simulink model "youBot_Arm_before_acceleration_test"  (R2024a)
settings: Solver=ode15s  StartTime=0.0  StopTime=3.3  MaxStep=1e-2  RelTol=1e-3  AbsTol=1e-4
model workspace: external: MATLAB File youBot_DataFile.m (data not in the file)
undefined symbols (not defined in the file): Extr_Data_LinkHoles, Qt, sigbuilder_block, smiData, X, Y, YBT_Par, Z
libraries: sm_lib x193, nesl_utility x130, fl_lib x53, simulink x13, Parts_Lib x10, MyMath_lib x8, Motor_Lib x5, Contact_Forces_Lib x4, ee_lib x2, sdl_lib x2
(part 1 of 8)
CloseFcn:
  | try,close(h1_youBot_Arm),end
  | clear h1_youBot_Arm
  | try,close(h2_youBot_Arm),end
  | clear h2_youBot_Arm
  | try,close(h3_youBot_Arm),end
  | clear h3_youBot_Arm
  | try,close(h4_youBot_Arm),end
  | clear h4_youBot_Arm
  | try,close(h5_youBot_Arm),end
  | clear h5_youBot_Arm
  | 
  | try,close(h1_youbot_optim),end
  | clear h1_youbot_optim
  | try,close(h2_youbot_optim),end
  | clear h2_youbot_optim
  | try,close(h3_youbot_optim),end
  | clear h3_youbot_optim
  | try,close(h4_youbot_optim),end
  | clear h4_youbot_optim
  | 
  | 
  | clear simlog_youBot_Arm
  | clear logsout_simlog_youBot_Arm
Description:
  | youBot Arm
  | 
  | Copyright 2017-2024 The MathWorks, Inc.
settings Model: Creator=smiller  LastModifiedBy=ADMIN
settings SolverCC: AutoScaleAbsTol=off  AlgebraicLoopSolver=TrustRegion
settings DataIOCC: MaxDataPoints=15000  ReturnWorkspaceOutputs=off  SignalLoggingName=logsout_youBot_Arm
settings OptimizationCC: ReuseModelBlockBuffer=off
settings DebuggingCC: UnconnectedInputMsg=warning  UnconnectedOutputMsg=warning  UnconnectedLineMsg=warning  PregeneratedLibrarySubsystemCodeDiagnostic=none  ArithmeticOperatorsInVariantConditions=warning
settings ModelReferenceCC: EnableRefExpFcnMdlSchedulingChecks=on
settings SFSimCC: SimUseLocalCustomCode=off  CustomCodeUndefinedFunction=UseInterfaceOnly
settings RTWCC: RTWUseLocalCustomCode=off  GPUComputeCapability=3.5  DLArmComputeVersion=19.05
settings CodeAppCC: StateflowObjectComments=on
settings SimscapeCC: SimscapeNormalizeSystem=off  SimscapeLogType=all  SimscapeLogSimulationStatistics=on  SimscapeLogName=simlog_youBot_Arm  SimscapeLogLimitData=off  SimscapeLogDataHistory=15000
settings DiagnosticsConfigSet: SimMechanicsUnconnectedFramePorts=none  SimMechanicsUnconnectedGeometryPorts=none  SimMechanicsRigidlyBoundBlock=none
settings ExplorerConfigSet: InternalSimMechanicsExplorerSettings="<ExplorerConfiguration><canonicalview>default</canonicalview><AnimationSetting><BasePlaybackSpeed>1.0</BasePlaybackSpeed><PlaybackSpeedFactor>1.0</PlaybackSpeedFactor></AnimationSetting><TilePanel><TileInfo><Tiles Columns=\"1\" Count=\"1\" Rows=\"1\"><Column Left=\"2\" Weight=\"1\"/><Column Left=\"827\"/><Row Top=\"2\" Weight=\"1\"/><Row Top=\"551\"/><Tile Height=\"1\" Width=\"1\" X=\"0\" Y=\"0\"/></Tiles></TileInfo><SceneInfo><SceneViewer><BGColor><R>1</R><G>1</G><B>1</B></BGColor><Camera><DoPerspective>off</DoPerspective><Position><X>-0.83626486692763047</X><Y>0.83378966470538818</Y><Z>0.42271625808458047</Z></Position><Center><X>-0.12358625191225214</X><Y>0.13538177403089358</Y><Z>0.35702295596507261</Z></Center><Up><X>0.049916044320742092</X><Y>-0.042921475658829755</Y><Z>0.99783071482423225</Z></Up><ViewLimDist>1</ViewLimDist><YLim>0.36726038306951525</YLim><XLim>0.55497124552726751</XLim></Camera></SceneViewer></SceneInfo></TilePanel><MechEditorPanel><Cameras><Camera><Id>Camera1</Id><Value><Name>Box Rear</Name><NativeCamera><PositionTrackingFeature>Arm.Environment.Load.Box.Camera_Frames.Box_Rear.F</PositionTrackingFeature><CenterTrackingFeature>Arm.Environment.Load.Box.Camera_Frames.Box_Rear.F</CenterTrackingFeature><UpVectorTrackingFeature>Arm.Base.B</UpVectorTrackingFeature><CenterTrackingOrigin>off</CenterTrackingOrigin><CenterTrackingDirection>-Y</CenterTrackingDirection><UpVectorTrackingDirection>+Z</UpVectorTrackingDirection></NativeCamera></Value></Camera><Camera><Id>Camera2</Id><Value><Name>Box Right</Name><NativeCamera><PositionTrackingFeature>Arm.Environment.Load.Box.Camera_Frames.Box_Right.F</PositionTrackingFeature><CenterTrackingFeature>Arm.Environment.Load.Box.Camera_Frames.Box_Right.F</CenterTrackingFeature><UpVectorTrackingFeature>Arm.Base.B</UpVectorTrackingFeature><CenterTrackingOrigin>off</CenterTrackingOrigin><CenterTrackingDirection>+X</CenterTrackingDirection><UpVectorTrackingDirection>+Z</UpVectorTrackingDirection></NativeCamera></Value></Camera><Camera><Id>Camera3</Id><Value><Name>Box Left</Name><NativeCamera><PositionTrackingFeature>Arm.Environment.Load.Box.Camera_Frames.Box_Left.F</PositionTrackingFeature><CenterTrackingFeature>Arm.Environment.Load.Box.Camera_Frames.Box_Left.F</CenterTrackingFeature><UpVectorTrackingFeature>Arm.Base.B</UpVectorTrackingFeature><CenterTrackingOrigin>off</CenterTrackingOrigin><CenterTrackingDirection>-X</CenterTrackingDirection><UpVectorTrackingDirection>+Z</UpVectorTrackingDirection></NativeCamera></Value></Camera><Camera><Id>Camera4</Id><Value><Name>Flythrough</Name><NativeCamera><PositionKeyframeSet><Keyframe><Time>+0.0000000000000000e+00</Time><Value><X>-3.1054174760408881e-01</X><Y>+1.3491196588304544e+00</Y><Z>+3.2708238484160229e-01</Z></Value></Keyframe><Keyframe><Time>+2.2800000000000002e+00</Time><Value><X>-3.1054175822801983e-01</X><Y>+1.3491196588304541e+00</Y><Z>+3.2708238484160196e-01</Z></Value></Keyframe><Keyframe><Time>+5.1399999999999997e+00</Time><Value><X>-4.2421722692384516e-03</X><Y>+3.7992130540546115e-01</Y><Z>+2.9693194824033292e-01</Z></Value></Keyframe><Keyframe><Time>+6.3200000000000003e+00</Time><Value><X>-4.2421722692384516e-03</X><Y>+3.7992130540546115e-01</Y><Z>+2.9693194824033292e-01</Z></Value></Keyframe><Keyframe><Time>+6.9600000000000000e+00</Time><Value><X>+4.9536995356902480e-04</X><Y>+4.7137606352469363e-01</Y><Z>+9.0060852468013763e-02</Z></Value></Keyframe><Keyframe><Time>+9.0400000000000009e+00</Time><Value><X>-3.5306739807128906e-01</X><Y>+1.4091664089762709e-01</Y><Z>+7.5516276061534882e-02</Z></Value></Keyframe><Keyframe><Time>+1.1180000000000000e+01</Time><Value><X>-3.5306739807128906e-01</X><Y>+1.4091664089762709e-01</Y><Z>+7.5516276061534882e-02</Z></Value></Keyframe><Keyframe><Time>+1.3280000000000001e+01</Time><Value><X>-7.3703070570058815e-01</X><Y>+4.8587438383396610e-02</Y><Z>+1.0735257722565938e-01</Z></Value></Keyframe><Keyframe><Time>+1.4180000000000000e+01</Time><Value><X>-7.3703070570058815e-01</X><Y>+4.8587438383396610e-02</Y><Z>+1.0735257722565938e-01</Z></Value></Keyframe><Keyframe><Time>+1.6520000000000000e+01</Time><Value><X>-9.8573824482540429e-01</X><Y>+2.0670485208261197e-01</Y><Z>+2.1830120652472185e-01</Z></Value></Keyframe></PositionKeyframeSet><CenterKeyframeSet><Keyframe><Time>+0.0000000000000000e+00</Time><Value><X>-3.1054174760408881e-01</X><Y>+6.2094819104938748e-01</Y><Z>+3.2708238484160207e-01</Z></Value></Keyframe><Keyframe><Time>+2.2800000000000002e+00</Time><Value><X>-3.1054175822801983e-01</X><Y>+6.2094819104938725e-01</Y><Z>+3.2708238484160190e-01</Z></Value></Keyframe><Keyframe><Time>+5.1399999999999997e+00</Time><Value><X>-4.2448177918945106e-03</X><Y>+3.8051098782519893e-01</Y><Z>+5.9999998663807202e-02</Z></Value></Keyframe><Keyframe><Time>+6.3200000000000003e+00</Time><Value><X>-4.2448177918945106e-03</X><Y>+3.8051098782519893e-01</Y><Z>+5.9999998663807147e-02</Z></Value></Keyframe><Keyframe><Time>+6.9600000000000000e+00</Time><Value><X>+4.9536995356902480e-04</X><Y>+6.2306314706802368e-02</Y><Z>+9.0060852468013763e-02</Z></Value></Keyframe><Keyframe><Time>+9.0400000000000009e+00</Time><Value><X>-3.5306739807128906e-01</X><Y>+3.5937078297138214e-02</Y><Z>+7.5516276061534882e-02</Z></Value></Keyframe><Keyframe><Time>+1.1180000000000000e+01</Time><Value><X>-3.5306739807128906e-01</X><Y>+1.6846667071218728e-02</Y><Z>+7.5516276061534854e-02</Z></Value></Keyframe><Keyframe><Time>+1.3280000000000001e+01</Time><Value><X>-2.6908442378044128e-01</X><Y>+4.8587438383396610e-02</Y><Z>+1.0735257722565938e-01</Z></Value></Keyframe><Keyframe><Time>+1.4180000000000000e+01</Time><Value><X>-2.0696524530649185e-02</X><Y>+4.8587438383396610e-02</Y><Z>+1.0735257722565938e-01</Z></Value></Keyframe><Keyframe><Time>+1.6520000000000000e+01</Time><Value><X>-4.4591089802364647e-01</X><Y>+2.0670485208261191e-01</Y><Z>+2.1830120652472185e-01</Z></Value></Keyframe></CenterKeyframeSet><UpVectorKeyframeSet><Keyframe><Time>+0.0000000000000000e+00</Time><Value><X>+0.0000000000000000e+00</X><Y>-0.0000000000000000e+00</Y><Z>+1.0000000000000000e+00</Z></Value></Keyframe><Keyframe><Time>+2.2800000000000002e+00</Time><Value><X>+0.0000000000000000e+00</X><Y>-0.0000000000000000e+00</Y><Z>+1.0000000000000000e+00</Z></Value></Keyframe><Keyframe><Time>+5.1399999999999997e+00</Time><Value><X>-1.1959347625026685e-03</X><Y>-9.9999618779192856e-01</Y><Z>-2.4888032573367248e-03</Z></Value></Keyframe><Keyframe><Time>+6.3200000000000003e+00</Time><Value><X>-1.1959347625026687e-03</X><Y>-9.9999618779192878e-01</Y><Z>-2.4888032573366957e-03</Z></Value></Keyframe><Keyframe><Time>+6.9600000000000000e+00</Time><Value><X>+0.0000000000000000e+00</X><Y>-0.0000000000000000e+00</Y><Z>+1.0000000000000000e+00</Z></Value></Keyframe><Keyframe><Time>+9.0400000000000009e+00</Time><Value><X>+0.0000000000000000e+00</X><Y>-0.0000000000000000e+00</Y><Z>+1.0000000000000000e+00</Z></Value></Keyframe><Keyframe><Time>+1.1180000000000000e+01</Time><Value><X>+0.0000000000000000e+00</X><Y>-0.0000000000000000e+00</Y><Z>+1.0000000000000000e+00</Z></Value></Keyframe><Keyframe><Time>+1.3280000000000001e+01</Time><Value><X>+0.0000000000000000e+00</X><Y>+0.0000000000000000e+00</Y><Z>+1.0000000000000000e+00</Z></Value></Keyframe><Keyframe><Time>+1.4180000000000000e+01</Time><Value><X>+0.0000000000000000e+00</X><Y>+0.0000000000000000e+00</Y><Z>+1.0000000000000000e+00</Z></Value></Keyframe><Keyframe><Time>+1.6520000000000000e+01</Time><Value><X>+0.0000000000000000e+00</X><Y>+0.0000000000000000e+00</Y><Z>+1.0000000000000000e+00</Z></Value></Keyframe></UpVectorKeyframeSet></NativeCamera></Value></Camera></Cameras><GfxPanelCameraMap/><VideoCreator><PlaybackSpeedRatio>1.0</PlaybackSpeedRatio><FrameRate>30</FrameRate><VideoFormat>MPEG-4</VideoFormat><FrameSize>auto</FrameSize></VideoCreator></MechEditorPanel></ExplorerConfiguration>"

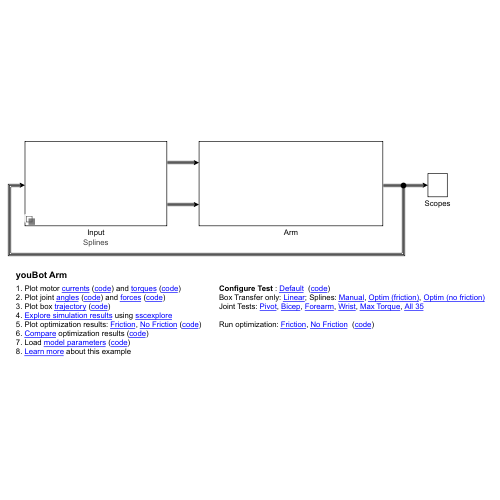
[thumbnail: Simulink's stored preview of the top-level diagram]
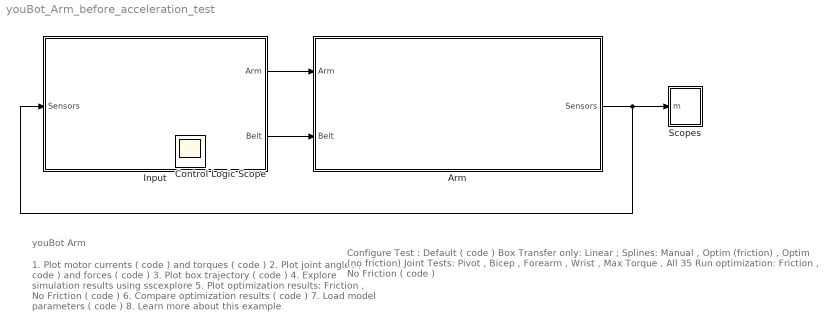
== system youBot_Arm_before_acceleration_test ==
  note: youBot Arm
  note: 1. Plot motor currents ( code ) and torques ( code )
      | 2. Plot joint angles ( code ) and forces ( code )
      | 3. Plot box trajectory ( code )
      | 4. Explore simulation results using sscexplore
      | 5. Plot optimization results: Friction , No Friction ( code )
      | 6. Compare optimization results ( code )
      | 7. Load model parameters ( code )
      | 8. Learn more about this example
  note: Configure Test : Default ( code )
      | Box Transfer only: Linear ; Splines: Manual , Optim (friction) , Optim (no friction)
      | Joint Tests: Pivot , Bicep , Forearm , Wrist , Max Torque , All 35
      |
      | Run optimization: Friction , No Friction ( code )
  Arm : Subsystem
      mask Display: image('youBot_Arm_System_IMAGE.jpg');
  Input : Subsystem  Tag=PublishSubsystem  Variant=on  VariantControlMode=label  VariantControl=Variant1  LabelModeActiveChoice=Splines
      settings: AttributesFormatString=%<ActiveVariant>
      mask Display:
      | blk = youBot_Arm_activeVariantBlock(gcb);
      | eval(get_param(blk, 'MaskDisplay'));
  Scopes : Subsystem
  Control Logic Scope : Scope
  wires:
  Input/1(Arm) -> Arm/1(Arm)
  Input/2(Belt) -> Arm/2(Belt)
  Arm/1(Sensors) -> Scopes/1(m), Input/1(Sensors)

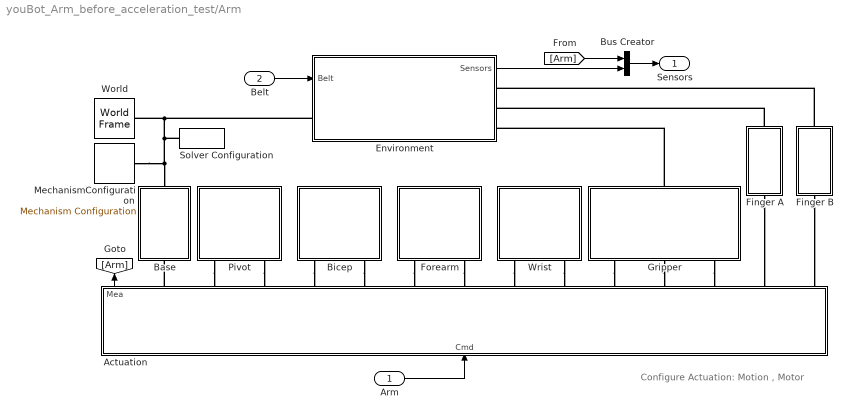
== system youBot_Arm_before_acceleration_test/Arm ==
  note: Configure Actuation: Motion , Motor
  Arm : Inport
  Belt : Inport  Port=2
  Actuation : Subsystem  Variant=on  VariantControlMode=label  LabelModeActiveChoice=Motion
      settings: AttributesFormatString=%<ActiveVariant>
      mask Display:
      | blk = youBot_Arm_activeVariantBlock(gcb);
      | eval(get_param(blk, 'MaskDisplay'));
  Base : Subsystem
      mask Display:
      | image('youBot_Arm_Base_IMAGE.jpg');
      | text(0.4,0.75,get_param(gcb,'Name'));
  Bicep : Subsystem
      mask Display:
      | image('youBot_Arm_Bicep_IMAGE.jpg');
      | text(0.6,0.9,get_param(gcb,'Name'));
  Bus Creator : BusCreator  Inputs=2
  Environment : Subsystem  Tag=PublishSubsystem
      mask Display: image('youBot_Arm_Environment_IMAGE.jpg');
  Finger A : Subsystem
      mask Display: image('youBot_Arm_Finger_A_IMAGE.jpg');
  Finger B : Subsystem
      mask Display: image('youBot_Arm_Finger_B_IMAGE.jpg');
  Forearm : Subsystem
      mask Display:
      | image('youBot_Arm_Forearm_IMAGE.jpg');
      | text(0.4,0.9,get_param(gcb,'Name'));
  Gripper : Subsystem
      mask Display:
      | image('youBot_Arm_Gripper_IMAGE.jpg');
      | text(0.6,0.9,'Gripper')
  MechanismConfiguration : sm_lib/Utilities/Mechanism Configuration  UniformGravity=Constant  GravityVector=[0 0 -9.81]  GravityVectorUnits=m/s^2  LinearizationDelta=0.001  JointModeTransitionNonlinearIterations=2
  Pivot : Subsystem
      mask Display:
      | image('youBot_Arm_Pivot_IMAGE.jpg');
      | text(0.6,0.9,get_param(gcb,'Name'));
  Solver Configuration : nesl_utility/Solver Configuration  PhysicalDomain=network_engine_domain  SubClassName=solver  LeftPortType=input  RightPortType=generic  Tones=[]  Harmonics=[]  SimulateNoise=off  Profile=off  UseLocalSampling=off  EnableSwitchedLinearOptims=on  FrequencyDomain=off  UseCCode=off  RelTol=0.001  AbsTol=1e-06  MinStep=1e-09  ToWorkspace=off  RevertToSquareIcSolve=off  NumHomotopyIterations=100  PhasorMode=off  PhasorModeNumHarmonics=1  ConsistencySolver=NEWTON_FTOL  IndexReductionMethod=DerivativeReplacement  DoDC=off  ResidualTolerance=1e-09  ConsistencyTolSource=GLOBAL  ConsistencyAbsTol=0.001  ConsistencyRelTol=0.001  ConsistencyTolFactor=0.001  UseLocalSolver=off  LocalSolverChoice=NE_BACKWARD_EULER_ADVANCER  ResolveIndetEquations=on  FunctionEvalNumThread=1  LocalSolverSampleTime=0.001  DoFixedCost=off  MaxNonlinIter=3  MaxModeIter=2  ComputeImpulses=off  ImpulseIterations=2  LinearAlgebra=Sparse  LinearAlgebraNumThread=0  EquationFormulation=NE_TIME_EF  DelaysMemoryBudget=1024  AutomaticFiltering=on  FilteringTimeConstant=0.001  PartitionStorageMethod=AS_NEEDED  PartitionMemoryBudget=1024  PartitionMethod=FAST  MultibodyUseLocalSolver=off  MultibodyLocalSolverChoice=ODE1  MultibodyLocalSolverSampleTime=0.001
  World : sm_lib/Frames and Transforms/World Frame
  Wrist : Subsystem
      mask Display:
      | image('youBot_Arm_Wrist_IMAGE.jpg');
      | text(0.6,0.9,get_param(gcb,'Name'));
  Sensors : Outport  VectorParamsAs1DForOutWhenUnconnected=off
  wires:
  Arm/1 -> Actuation/1(Cmd)
  Actuation/1(Mea) -> [Arm]
  Belt/1 -> Environment/1(Belt)
  Environment/1(Sensors) -> Bus Creator/2
  [Arm] -> Bus Creator/1
  Bus Creator/1 -> Sensors/1
  connections:
  Pivot/RConn1 -- Actuation/RConn2
  Wrist/RConn3 -- Actuation/RConn9
  Forearm/RConn1 -- Actuation/RConn6
  Forearm/RConn3 -- Actuation/RConn7
  Wrist/RConn1 -- Actuation/RConn8
  Pivot/RConn3 -- Actuation/RConn3
  Bicep/RConn1 -- Actuation/RConn4
  Bicep/RConn3 -- Actuation/RConn5
  Gripper/RConn1 -- Actuation/RConn10
  Finger A/LConn1 -- Actuation/RConn13
  Gripper/RConn3 -- Actuation/RConn12
  Gripper/RConn2 -- Actuation/RConn11
  Finger B/LConn1 -- Actuation/RConn14
  Actuation/RConn1 -- Base/RConn1
  MechanismConfiguration/RConn1 -- Environment/LConn1 -- World/RConn1 -- Solver Configuration/RConn1 -- Base/LConn1
  Finger B/RConn1 -- Environment/RConn1
  Finger A/RConn1 -- Environment/RConn2
  Gripper/LConn1 -- Environment/RConn3

== system youBot_Arm_before_acceleration_test/Input ==
  Sensors : Inport
  Control : Subsystem  VariantControl=Control
      mask Display:
      | image('youBot_Arm_Input_Control_IMAGE.jpg');
      | text(0.43,0.7,'Home');
      | text(0.235,0.32,'Belt In');
      | text(0.59,0.32,'Belt Out');
  Control Belt : Subsystem  VariantControl=Control_Belt
      mask Display:
      | image('youBot_Arm_Input_Control_Belt_IMAGE.jpg');
      | text(0.44,0.26,'Belts');
  Signals : Subsystem  VariantControl=Signals
      mask Display:
      | image('youBot_Arm_Input_Signals_IMAGE.jpg');
      | [~, activeGroupLabel]= signalbuilder([bdroot '/Input/Signals/Robot Commands'], 'activegroup');
      | text(0.25,0.5,activeGroupLabel);
  Splines : Subsystem  VariantControl=Splines
      mask Display: image('youBot_Arm_Input_Splines_IMAGE.jpg');
  Arm : Outport  VectorParamsAs1DForOutWhenUnconnected=off
  Belt : Outport  Port=2  VectorParamsAs1DForOutWhenUnconnected=off

== system youBot_Arm_before_acceleration_test/Scopes ==
  m : Inport
  Bus Selector : BusSelector  OutputSignals=Arm.P.t,Arm.B.t,Arm.F.t,Arm.W.t,Arm.G.t,Arm.a.f,Arm.b.f
  Bus Selector1 : BusSelector  OutputSignals=Arm.P.i,Arm.B.i,Arm.F.i,Arm.W.i,Arm.G.i,Arm.a.i,Arm.b.i
  Calculate Electrical Cost : Subsystem
  Calculate Torque Cost : Subsystem
  Currents : Scope  NumInputPorts=7
  Display : Display
  Display1 : Display
  Logging : Subsystem
  Mux : Mux
  Mux1 : Mux  Inputs=7
  Selector : Selector  InputPortWidth=7  IndexOptions=Index vector (dialog)  Indices=[1:4]  OutputSizes=1
  Terminator : Terminator
  Terminator1 : Terminator
  Torques : Scope  NumInputPorts=7
  wires:
  m/1 -> Bus Selector/1, Bus Selector1/1, Logging/1(In1)
  Bus Selector/1 -> Mux/1, Torques/1  "<t>"
  Bus Selector/2 -> Mux/2, Torques/2  "<t>"
  Bus Selector/4 -> Mux/4, Torques/4  "<t>"
  Bus Selector/7 -> Torques/7  "<f>"
  Bus Selector/3 -> Mux/3, Torques/3  "<t>"
  Bus Selector/5 -> Torques/5  "<t>"
  Bus Selector/6 -> Torques/6  "<f>"
  Mux/1 -> Calculate Torque Cost/1(x)
  Calculate Torque Cost/1(Int(x'*x)) -> Display/1, Terminator/1
  Bus Selector1/5 -> Mux1/5, Currents/5  "<i>"
  Bus Selector1/6 -> Mux1/6, Currents/6  "<i>"
  Bus Selector1/7 -> Mux1/7, Currents/7  "<i>"
  Bus Selector1/3 -> Mux1/3, Currents/3  "<i>"
  Bus Selector1/2 -> Mux1/2, Currents/2  "<i>"
  Bus Selector1/1 -> Mux1/1, Currents/1  "<i>"
  Bus Selector1/4 -> Mux1/4, Currents/4  "<i>"
  Mux1/1 -> Selector/1
  Calculate Electrical Cost/1(Int(x'*x)) -> Terminator1/1, Display1/1
  Selector/1 -> Calculate Electrical Cost/1(i)

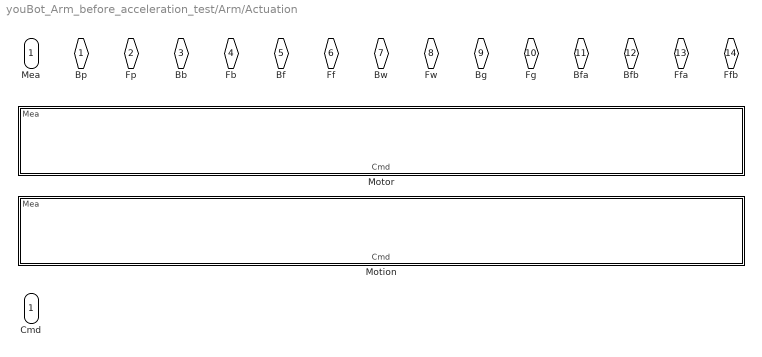
== system youBot_Arm_before_acceleration_test/Arm/Actuation ==
  Cmd : Inport
  Motion : Subsystem  Tag=PublishSubsystem  VariantControl=Motion
      mask Display: image('youBot_Arm_Actuation_Motion_IMAGE.jpg');
  Motor : Subsystem  Tag=PublishSubsystem  VariantControl=Motor
      mask Display: image('youBot_Arm_Actuation_Motor_IMAGE.jpg');
  Bp : PMIOPort  Side=Right
  Fp : PMIOPort  Port=2  Side=Right
  Bb : PMIOPort  Port=3  Side=Right
  Fb : PMIOPort  Port=4  Side=Right
  Bf : PMIOPort  Port=5  Side=Right
  Ff : PMIOPort  Port=6  Side=Right
  Bw : PMIOPort  Port=7  Side=Right
  Fw : PMIOPort  Port=8  Side=Right
  Bg : PMIOPort  Port=9  Side=Right
  Fg : PMIOPort  Port=10  Side=Right
  Bfa : PMIOPort  Port=11  Side=Right
  Bfb : PMIOPort  Port=12  Side=Right
  Ffa : PMIOPort  Port=13  Side=Right
  Ffb : PMIOPort  Port=14  Side=Right
  Mea : Outport  VectorParamsAs1DForOutWhenUnconnected=off

== system youBot_Arm_before_acceleration_test/Arm/Base ==
  Base_1_RIGID : Subsystem
  Transform : sm_lib/Frames and Transforms/Rigid Transform  RotationMethod=ArbitraryAxis  FollAlignAxisA=+X  BaseAlignAxisA=+Y  FollAlignAxisB=+Y  BaseAlignAxisB=+Z  RotationStandardAxis=+Z  RotationAngle=smiData.RigidTransform(49).angle  RotationAngleUnits=rad  RotationArbitraryAxis=smiData.RigidTransform(49).axis  RotationSequenceAxes=FollowerAxes  RotationSequence=XYX  RotationSequenceAngles=[0 0 0]  RotationSequenceAnglesUnits=deg  RotationMatrix=[1 0 0; 0 1 0; 0 0 1]  Quaternion=[1 0 0 0]  TranslationMethod=Cartesian  TranslationCartesianOffset=smiData.RigidTransform(49).translation  TranslationCartesianOffsetUnits=m  TranslationStandardAxis=+Z  TranslationStandardOffset=0  TranslationStandardOffsetUnits=m  TranslationROffset=0  TranslationROffsetUnits=m  TranslationThetaOffset=0  TranslationThetaOffsetUnits=deg  TranslationZOffset=0  TranslationZOffsetUnits=m
  B : PMIOPort  Side=Left
  F : PMIOPort  Port=2  Side=Right
  connections:
  Base_1_RIGID/RConn1 -- F/RConn1
  Transform/LConn1 -- B/RConn1
  Base_1_RIGID/LConn1 -- Transform/RConn1

== system youBot_Arm_before_acceleration_test/Arm/Bicep ==
  note: Connection 2 added only to adjust position of subsystem ports.
  Bicep_1_RIGID : Subsystem
  B : PMIOPort  Side=Right
  ~ : PMIOPort  Tag=CustomStyle  Port=2  Side=Right
  F : PMIOPort  Port=3  Side=Right
  connections:
  Bicep_1_RIGID/LConn1 -- B/RConn1
  ~/RConn1 -- Bicep_1_RIGID/RConn1 -- F/RConn1

== system youBot_Arm_before_acceleration_test/Arm/Environment ==
  note: Configure Load: Payload , Damper , Penalty
  Belt : Inport
  Conveyors : Subsystem
      mask Display: image('youBot_Arm_Conveyors_IMAGE.jpg');
  EE Signals : Subsystem
  Floor : Subsystem
  Gripper Force : Subsystem  Tag=PublishSubsystem  Variant=on  VariantControlMode=label  LabelModeActiveChoice=Payload
      settings: AttributesFormatString=%<ActiveVariant>
      mask Display:
      | blk = youBot_Arm_activeVariantBlock(gcb);
      | eval(get_param(blk, 'MaskDisplay'));
  Load : Subsystem  Variant=on  VariantControlMode=label  LabelModeActiveChoice=None
      settings: AttributesFormatString=%<ActiveVariant>
      mask Display:
      | blk = youBot_Arm_activeVariantBlock(gcb);
      | eval(get_param(blk, 'MaskDisplay'));
  To Workspace : ToWorkspace  VariableName=EE_xyz  SaveFormat=Structure With Time  SampleTime=-1
  Transform Sensor EE : sm_lib/Frames and Transforms/Transform Sensor  MeasurementFrame=World  RotationSequence=XYX  SenseAngle=off  SenseAxis=off  SenseQ=off  SenseR=off  SenseRotationSequence=off  SenseOmegaX=off  SenseOmegaY=off  SenseOmegaZ=off  SenseOmega=off  SenseQDot=off  SenseRDot=off  SenseRotationSequenceDot=off  SenseAlphaX=off  SenseAlphaY=off  SenseAlphaZ=off  SenseAlpha=off  SenseQDDot=off  SenseRDDot=off  SenseX=on  SenseY=on  SenseZ=on  SenseXYZ=off  SenseRad=off  SenseAzim=off  SenseDist=off  SenseInc=off  SenseXDot=off  SenseYDot=off  SenseZDot=off  SenseXYZDot=off  SenseRadDot=off  SenseAzimDot=off  SenseDistDot=off  SenseIncDot=off  SenseXDDot=off  SenseYDDot=off  SenseZDDot=off  SenseXYZDDot=off  SenseRadDDot=off  SenseAzimDDot=off  SenseDistDDot=off  SenseIncDDot=off
  W : PMIOPort  Side=Left
  Fb : PMIOPort  Port=2  Side=Right
  Fa : PMIOPort  Port=3  Side=Right
  E : PMIOPort  Port=4  Side=Right
  Sensors : Outport  VectorParamsAs1DForOutWhenUnconnected=off
  wires:
  EE Signals/1(xyz) -> To Workspace/1
  Belt/1 -> Conveyors/1(Belt)
  Conveyors/1(Sensors) -> Sensors/1
  connections:
  Gripper Force/RConn1 -- Fa/RConn1
  Gripper Force/LConn1 -- Load/RConn1
  Gripper Force/RConn3 -- Fb/RConn1
  Gripper Force/LConn2 -- Load/RConn2
  Gripper Force/RConn2 -- Transform Sensor EE/RConn1 -- E/RConn1
  EE Signals/LConn1 -- Transform Sensor EE/RConn2
  EE Signals/LConn2 -- Transform Sensor EE/RConn3
  EE Signals/LConn3 -- Transform Sensor EE/RConn4
  Load/LConn1 -- Conveyors/RConn1
  Load/LConn2 -- Transform Sensor EE/LConn1 -- Floor/LConn1 -- W/RConn1 -- Conveyors/LConn1

== system youBot_Arm_before_acceleration_test/Arm/Finger A ==
  Finger_A_1_RIGID : Subsystem
  F : PMIOPort  Side=Left
  f : PMIOPort  Port=2  Side=Right
  connections:
  f/RConn1 -- Finger_A_1_RIGID/RConn1
  F/RConn1 -- Finger_A_1_RIGID/LConn1

== system youBot_Arm_before_acceleration_test/Arm/Finger B ==
  Finger_B_1_RIGID : Subsystem
  F : PMIOPort  Side=Left
  f : PMIOPort  Port=2  Side=Right
  connections:
  f/RConn1 -- Finger_B_1_RIGID/RConn1
  Finger_B_1_RIGID/LConn1 -- F/RConn1

== system youBot_Arm_before_acceleration_test/Arm/Forearm ==
  note: Connection 2 added only to adjust position of subsystem ports.
  Forearm_1_RIGID : Subsystem
  Forearm_Black_Inlay_1_RIGID : Subsystem
  B : PMIOPort  Side=Right
  ~ : PMIOPort  Port=2  Side=Right
  F : PMIOPort  Port=3  Side=Right
  connections:
  Forearm_1_RIGID/LConn2 -- B/RConn1
  ~/RConn1 -- Forearm_1_RIGID/RConn1 -- F/RConn1
  Forearm_1_RIGID/LConn1 -- Forearm_Black_Inlay_1_RIGID/LConn1

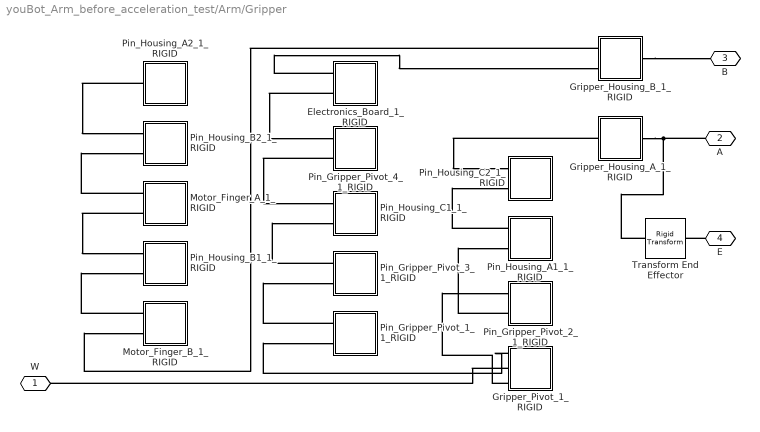
== system youBot_Arm_before_acceleration_test/Arm/Gripper ==
  Electronics_Board_1_RIGID : Subsystem
  Gripper_Housing_A_1_RIGID : Subsystem
  Gripper_Housing_B_1_RIGID : Subsystem
  Gripper_Pivot_1_RIGID : Subsystem
  Motor_Finger_A_1_RIGID : Subsystem
  Motor_Finger_B_1_RIGID : Subsystem
  Pin_Gripper_Pivot_1_1_RIGID : Subsystem
  Pin_Gripper_Pivot_2_1_RIGID : Subsystem
  Pin_Gripper_Pivot_3_1_RIGID : Subsystem
  Pin_Gripper_Pivot_4_1_RIGID : Subsystem
  Pin_Housing_A1_1_RIGID : Subsystem
  Pin_Housing_A2_1_RIGID : Subsystem
  Pin_Housing_B1_1_RIGID : Subsystem
  Pin_Housing_B2_1_RIGID : Subsystem
  Pin_Housing_C1_1_RIGID : Subsystem
  Pin_Housing_C2_1_RIGID : Subsystem
  Transform End Effector : sm_lib/Frames and Transforms/Rigid Transform  RotationMethod=AlignedAxes  FollAlignAxisA=+Z  BaseAlignAxisA=-Z  FollAlignAxisB=+X  BaseAlignAxisB=+Y  RotationStandardAxis=+Z  RotationAngle=0.0  RotationAngleUnits=deg  RotationArbitraryAxis=[0 0 1]  RotationSequenceAxes=FollowerAxes  RotationSequence=XYX  RotationSequenceAngles=[0 0 0]  RotationSequenceAnglesUnits=deg  RotationMatrix=[1 0 0; 0 1 0; 0 0 1]  Quaternion=[1 0 0 0]  TranslationMethod=StandardAxis  TranslationCartesianOffset=[0 0 0]  TranslationCartesianOffsetUnits=m  TranslationStandardAxis=+X  TranslationStandardOffset=YBT_Par.Payload.gripper_ref_offset  TranslationStandardOffsetUnits=m  TranslationROffset=0  TranslationROffsetUnits=m  TranslationThetaOffset=0  TranslationThetaOffsetUnits=deg  TranslationZOffset=0  TranslationZOffsetUnits=m
  W : PMIOPort  Side=Right
  A : PMIOPort  Port=2  Side=Right
  B : PMIOPort  Port=3  Side=Right
  E : PMIOPort  Port=4  Side=Left
  connections:
  Gripper_Housing_B_1_RIGID/RConn1 -- B/RConn1
  A/RConn1 -- Gripper_Housing_A_1_RIGID/RConn1 -- Transform End Effector/LConn1
  E/RConn1 -- Transform End Effector/RConn1
  Pin_Gripper_Pivot_1_1_RIGID/LConn1 -- Pin_Gripper_Pivot_3_1_RIGID/LConn2
  Pin_Housing_A2_1_RIGID/LConn1 -- Pin_Housing_B2_1_RIGID/LConn1
  Gripper_Pivot_1_RIGID/LConn2 -- W/RConn1
  Gripper_Pivot_1_RIGID/LConn3 -- Pin_Gripper_Pivot_2_1_RIGID/LConn1
  Gripper_Pivot_1_RIGID/LConn1 -- Pin_Gripper_Pivot_1_1_RIGID/LConn2
  Pin_Housing_A1_1_RIGID/LConn1 -- Pin_Housing_C2_1_RIGID/LConn2
  Gripper_Housing_A_1_RIGID/LConn1 -- Pin_Housing_C2_1_RIGID/LConn1
  Motor_Finger_A_1_RIGID/LConn2 -- Pin_Housing_B1_1_RIGID/LConn1
  Gripper_Housing_B_1_RIGID/LConn1 -- Motor_Finger_B_1_RIGID/LConn2
  Electronics_Board_1_RIGID/LConn2 -- Pin_Gripper_Pivot_4_1_RIGID/LConn1
  Motor_Finger_A_1_RIGID/LConn1 -- Pin_Housing_B2_1_RIGID/LConn2
  Pin_Gripper_Pivot_3_1_RIGID/LConn1 -- Pin_Housing_C1_1_RIGID/LConn2
  Electronics_Board_1_RIGID/LConn1 -- Gripper_Housing_B_1_RIGID/LConn2
  Pin_Gripper_Pivot_2_1_RIGID/LConn2 -- Pin_Housing_A1_1_RIGID/LConn2
  Pin_Gripper_Pivot_4_1_RIGID/LConn2 -- Pin_Housing_C1_1_RIGID/LConn1
  Motor_Finger_B_1_RIGID/LConn1 -- Pin_Housing_B1_1_RIGID/LConn2

== system youBot_Arm_before_acceleration_test/Arm/Pivot ==
  note: Connection 2 added only to adjust position of subsystem ports.
  Pivot_1_RIGID : Subsystem
  Pivot_Black_Inlay_1_RIGID : Subsystem
  B : PMIOPort  Side=Right
  ~ : PMIOPort  Tag=CustomStyle  Port=2  Side=Right
  F : PMIOPort  Port=3  Side=Right
  connections:
  Pivot_1_RIGID/LConn2 -- B/RConn1
  ~/RConn1 -- Pivot_1_RIGID/RConn1 -- F/RConn1
  Pivot_1_RIGID/LConn1 -- Pivot_Black_Inlay_1_RIGID/LConn1

== system youBot_Arm_before_acceleration_test/Arm/Wrist ==
  note: Connection 2 added only to adjust position of subsystem ports.
  Wrist_1_RIGID : Subsystem
  B : PMIOPort  Side=Right
  ~ : PMIOPort  Port=2  Side=Right
  F : PMIOPort  Port=3  Side=Right
  connections:
  F/RConn1 -- ~/RConn1 -- Wrist_1_RIGID/RConn1
  Wrist_1_RIGID/LConn1 -- B/RConn1

== system youBot_Arm_before_acceleration_test/Input/Control ==
  Sensors : Inport
  Bus Creator : BusCreator  Inputs=2
  Bus Selector : BusSelector  OutputSignals=Belts.BeltIn.Box,Belts.BeltIn.LC,Belts.BeltOut.Box,Belts.BeltOut.LC
  Joint Commands : Subsystem  mask{home2in=YBT_Par.Waypoints.Home2In.Manual, in2out=YBT_Par.Waypoints.In2Out.Manual, out2home=YBT_Par.Waypoints.Out2Home.Manual}
      mask prompts: home2in "Home to Belt In"; in2out "Belt In to Belt Out"; out2home "Belt Out to Home"
  Logging : Subsystem
  Logic : Stateflow chart  Tag=PublishSubsystem  TreatAsAtomicUnit=on  mask(Supervisory Logic for Arm, Gripper, and Belts){delayMoveBox=YBT_Par.Control.Logic.Delay_Move_Box, delayGripBox=YBT_Par.Control.Logic.Delay_Grip_Box, delayDropBox=YBT_Par.Control.Logic.Delay_Drop_Box, delayClose=YBT_Par.Control.Logic.Delay_Close_Grip, delayBeltClear=YBT_Par.Control.Logic.Delay_Belt_Clear, delayShipBox=YBT_Par.Control.Logic.Delay_Ship_Box}
      mask prompts: delayMoveBox "Delay Move Box (sec)"; delayGripBox "Delay Grip Box (sec)"; delayDropBox "Delay Drop Box (sec)"; delayClose "Delay Close Gripper at Home (sec)"; delayBeltClear "Delay Belt Clear (sec)"; delayShipBox "Delay Ship Box (sec)"
      mask help: Logic controlling robot arm, gripper, and belts. Arm movement, gripper state, and belt state are controlled based on events in the system. The parameters below are for delays that ensure actions are not triggered too early.
  Arm : Outport  VectorParamsAs1DForOutWhenUnconnected=off
  Belt : Outport  Port=2  VectorParamsAs1DForOutWhenUnconnected=off
  wires:
  Bus Creator/1 -> Belt/1
  Bus Selector/4 -> Logic/4(BeltOut_LC)  "<LC>"
  Bus Selector/3 -> Logic/3(BeltOut_Box)  "<Box>"
  Bus Selector/2 -> Logic/2(BeltIn_LC)  "<LC>"
  Bus Selector/1 -> Logic/1(BeltIn_Box)  "<Box>"
  Sensors/1 -> Logging/1(S), Bus Selector/1
  Logic/3(BeltIn_En) -> Bus Creator/1  "Belt In On"
  Logic/1(Way) -> Joint Commands/1(Way)  "Way"
  Logic/2(Grip) -> Joint Commands/2(Grip)  "Grip"
  Logic/4(BeltOut_En) -> Bus Creator/2  "Belt Out On"
  Joint Commands/1(bus) -> Arm/1

== system youBot_Arm_before_acceleration_test/Input/Control Belt ==
  Sensors : Inport
  Bus Creator : BusCreator  Inputs=2
  Bus Selector : BusSelector  OutputSignals=Belts.BeltIn.Box,Belts.BeltIn.LC,Belts.BeltOut.Box,Belts.BeltOut.LC
  Control Belt In : Subsystem
  Control Belt Out : Subsystem
  Robot Commands : Subsystem  Tag=STV Subsys  LoadFcn=sigbuilder_block('load');  StartFcn=sigbuilder_block('start');  StopFcn=sigbuilder_block('stop');  ClipboardFcn=sigbuilder_block('clipboard');  mask(Sigbuilder block){tuvar=[0:10]}
      mask help: Simulink:masks:SigbuilderBlock_MD
      mask init:
      | if ~strcmp(get_param(bdroot(gcbh),'SimulationStatus'),'stopped') tuvar = sigbuilder_block('maskInit'); end
      settings: CopyFcn=sigbuilder_block('copy');  DeleteFcn=sigbuilder_block('delete');  ModelCloseFcn=sigbuilder_block('modelClose');  PreSaveFcn=sigbuilder_block('preSave');  PauseFcn=sigbuilder_block('pause');  ContinueFcn=sigbuilder_block('continue');  NameChangeFcn=sigbuilder_block('namechange');  OpenFcn=sigbuilder_block('open',[0 142.8 450.6 439.8 ]);  CloseFcn=sigbuilder_block('close');
      mask Display: plot(0, 0, 100, 100,[2, 2, 32, 32, 2], [68, 8, 8, 68, 68],[32, 2], [38, 38], [32, 19, 2],[53, 60, 44], [32, 17, 17, 2],[16, 16, 31, 31]);txt = getActiveGroup(gcbh);text(2, 100, txt,'verticalAlignment', 'top');
  Arm : Outport  VectorParamsAs1DForOutWhenUnconnected=off
  Belt : Outport  Port=2  VectorParamsAs1DForOutWhenUnconnected=off
  wires:
  Robot Commands/1(Bus) -> Arm/1
  Sensors/1 -> Bus Selector/1
  Bus Selector/1 -> Control Belt In/1(BeltOut)  "<Box>"
  Bus Selector/2 -> Control Belt In/2(Sensor)  "<LC>"
  Bus Selector/3 -> Control Belt Out/1(BeltOut)  "<Box>"
  Bus Selector/4 -> Control Belt Out/2(Sensor)  "<LC>"
  Control Belt In/1(On) -> Bus Creator/1  "Belt In On"
  Control Belt Out/1(On) -> Bus Creator/2  "Belt Out On"
  Bus Creator/1 -> Belt/1

== system youBot_Arm_before_acceleration_test/Input/Signals ==
  Belt Commands : Subsystem  Tag=STV Subsys  LoadFcn=sigbuilder_block('load');  StartFcn=sigbuilder_block('start');  StopFcn=sigbuilder_block('stop');  ClipboardFcn=sigbuilder_block('clipboard');  mask(Sigbuilder block){tuvar=[0:10]}
      mask help: Simulink:masks:SigbuilderBlock_MD
      mask init:
      | if ~strcmp(get_param(bdroot(gcbh),'SimulationStatus'),'stopped') tuvar = sigbuilder_block('maskInit'); end
      settings: CopyFcn=sigbuilder_block('copy');  DeleteFcn=sigbuilder_block('delete');  ModelCloseFcn=sigbuilder_block('modelClose');  PreSaveFcn=sigbuilder_block('preSave');  PauseFcn=sigbuilder_block('pause');  ContinueFcn=sigbuilder_block('continue');  NameChangeFcn=sigbuilder_block('namechange');  OpenFcn=sigbuilder_block('open',[19.2 172.2 550.8 400.2 ]);  CloseFcn=sigbuilder_block('close');
      mask Display: plot(0, 0, 100, 100,[2, 2, 32, 32, 2], [68, 8, 8, 68, 68],[32, 2], [38, 38], [32, 19, 2],[53, 60, 44], [32, 17, 17, 2],[16, 16, 31, 31]);txt = getActiveGroup(gcbh);text(2, 100, txt,'verticalAlignment', 'top');
  Robot Commands : Subsystem  Tag=STV Subsys  LoadFcn=sigbuilder_block('load');  StartFcn=sigbuilder_block('start');  StopFcn=sigbuilder_block('stop');  ClipboardFcn=sigbuilder_block('clipboard');  mask(Sigbuilder block){tuvar=[0:10]}
      mask help: Simulink:masks:SigbuilderBlock_MD
      mask init:
      | if ~strcmp(get_param(bdroot(gcbh),'SimulationStatus'),'stopped') tuvar = sigbuilder_block('maskInit'); end
      settings: CopyFcn=sigbuilder_block('copy');  DeleteFcn=sigbuilder_block('delete');  ModelCloseFcn=sigbuilder_block('modelClose');  PreSaveFcn=sigbuilder_block('preSave');  PauseFcn=sigbuilder_block('pause');  ContinueFcn=sigbuilder_block('continue');  NameChangeFcn=sigbuilder_block('namechange');  OpenFcn=sigbuilder_block('open',[0.6 142.2 450.6 439.8 ]);  CloseFcn=sigbuilder_block('close');
      mask Display: plot(0, 0, 100, 100,[2, 2, 32, 32, 2], [68, 8, 8, 68, 68],[32, 2], [38, 38], [32, 19, 2],[53, 60, 44], [32, 17, 17, 2],[16, 16, 31, 31]);txt = getActiveGroup(gcbh);text(2, 100, txt,'verticalAlignment', 'top');
  Arm : Outport  VectorParamsAs1DForOutWhenUnconnected=off
  Belt : Outport  Port=2  VectorParamsAs1DForOutWhenUnconnected=off
  wires:
  Robot Commands/1(Bus) -> Arm/1
  Belt Commands/1(Bus) -> Belt/1

== system youBot_Arm_before_acceleration_test/Input/Splines ==
  Bus Creator : BusCreator  Inputs=7
  Bus Creator3 : BusCreator  Inputs=2
  Clock : Clock
  Constant : Constant  Value=0
  Constant1 : Constant  Value=YBT_Par.Gripper.Position.tight
  Constant2 : Constant  Value=YBT_Par.Gripper.Position.tight
  Spline Bicep Angle : Lookup_n-D  NumberOfTableDimensions=1  LookupTableObject=''  BreakpointsForDimension1=t  Table=Qt(2,:)  InterpMethod=Cubic spline  ExtrapMethod=Clip  InternalRulePriority=Speed  RndMeth=Simplest
  Spline Forearm Angle : Lookup_n-D  NumberOfTableDimensions=1  LookupTableObject=''  BreakpointsForDimension1=t  Table=Qt(3,:)  InterpMethod=Cubic spline  ExtrapMethod=Clip  InternalRulePriority=Speed  RndMeth=Simplest
  Spline Pivot Angle : Lookup_n-D  NumberOfTableDimensions=1  LookupTableObject=''  BreakpointsForDimension1=t  Table=Qt(1,:)  InterpMethod=Cubic spline  ExtrapMethod=Clip  InternalRulePriority=Speed  RndMeth=Simplest
  Spline Wrist Angle : Lookup_n-D  NumberOfTableDimensions=1  LookupTableObject=''  BreakpointsForDimension1=t  Table=Qt(4,:)  InterpMethod=Cubic spline  ExtrapMethod=Clip  InternalRulePriority=Speed  RndMeth=Simplest
  vx : Constant  Value=0
  vy : Constant  Value=0
  Arm : Outport  VectorParamsAs1DForOutWhenUnconnected=off
  Belt : Outport  Port=2  VectorParamsAs1DForOutWhenUnconnected=off
  wires:
  Bus Creator/1 -> Arm/1
  Spline Pivot Angle/1 -> Bus Creator/1  "cP"
  Spline Bicep Angle/1 -> Bus Creator/2  "cB"
  Spline Forearm Angle/1 -> Bus Creator/3  "cF"
  Spline Wrist Angle/1 -> Bus Creator/4  "cW"
  Constant/1 -> Bus Creator/5  "cG"
  Constant1/1 -> Bus Creator/6  "ca"
  Constant2/1 -> Bus Creator/7  "cb"
  Clock/1 -> Spline Wrist Angle/1, Spline Forearm Angle/1, Spline Pivot Angle/1, Spline Bicep Angle/1
  vx/1 -> Bus Creator3/1  "Belt In On"
  vy/1 -> Bus Creator3/2  "Belt Out On"
  Bus Creator3/1 -> Belt/1

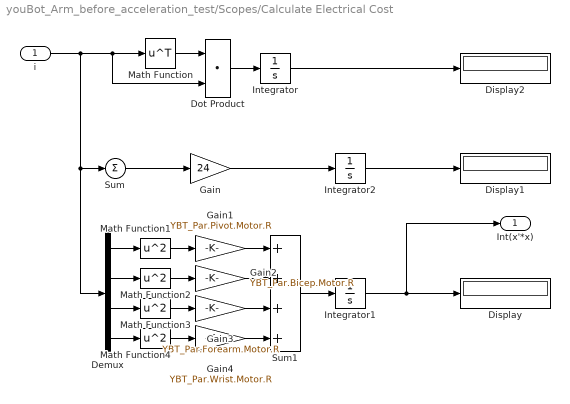
== system youBot_Arm_before_acceleration_test/Scopes/Calculate Electrical Cost ==
  i : Inport
  Demux : Demux
  Display : Display
  Display1 : Display
  Display2 : Display
  Dot Product : DotProduct  OutDataTypeStr=Inherit: Inherit via internal rule
  Gain : Gain  Gain=24
  Gain1 : Gain  Gain=YBT_Par.Pivot.Motor.R
  Gain2 : Gain  Gain=YBT_Par.Bicep.Motor.R
  Gain3 : Gain  Gain=YBT_Par.Forearm.Motor.R
  Gain4 : Gain  Gain=YBT_Par.Wrist.Motor.R
  Integrator : Integrator
  Integrator1 : Integrator
  Integrator2 : Integrator
  Math Function : Math  Operator=transpose  SignedPower=on
  Math Function{1..4} (4 alike) : Math  Operator=square  SignedPower=on
  Sum : Sum  Inputs=+
  Sum1 : Sum  Inputs=++++
  Int(x'*x) : Outport  VectorParamsAs1DForOutWhenUnconnected=off
  wires:
  Integrator/1 -> Display2/1
  i/1 -> Demux/1, Sum/1, Math Function/1, Dot Product/2
  Math Function/1 -> Dot Product/1
  Dot Product/1 -> Integrator/1
  Sum/1 -> Gain/1
  Demux/1 -> Math Function1/1
  Math Function1/1 -> Gain1/1
  Demux/2 -> Math Function2/1
  Math Function2/1 -> Gain2/1
  Demux/3 -> Math Function3/1
  Math Function3/1 -> Gain3/1
  Demux/4 -> Math Function4/1
  Math Function4/1 -> Gain4/1
  Gain1/1 -> Sum1/1
  Gain2/1 -> Sum1/2
  Gain3/1 -> Sum1/3
  Gain4/1 -> Sum1/4
  Sum1/1 -> Integrator1/1
  Gain/1 -> Integrator2/1
  Integrator1/1 -> Int(x'*x)/1, Display/1
  Integrator2/1 -> Display1/1

== system youBot_Arm_before_acceleration_test/Scopes/Calculate Torque Cost ==
  x : Inport
  Dot Product : DotProduct  OutDataTypeStr=Inherit: Inherit via internal rule
  Integrator : Integrator
  Math Function : Math  Operator=transpose  SignedPower=on
  Int(x'*x) : Outport  VectorParamsAs1DForOutWhenUnconnected=off
  wires:
  Dot Product/1 -> Integrator/1
  Math Function/1 -> Dot Product/1
  x/1 -> Dot Product/2, Math Function/1
  Integrator/1 -> Int(x'*x)/1

== system youBot_Arm_before_acceleration_test/Scopes/Logging ==
  In1 : Inport
  Log Constraint Forces : Subsystem
  Log Joint Angles : Subsystem
  Log Torques : Subsystem
  Terminator1 : Terminator
  Terminator2 : Terminator
  Terminator3 : Terminator
  wires:
  Log Torques/1(Out1) -> Terminator2/1
  Log Joint Angles/1(Out1) -> Terminator3/1
  In1/1 -> Log Constraint Forces/1(In1), Log Joint Angles/1(In1), Log Torques/1(In1)
  Log Constraint Forces/1(Out1) -> Terminator1/1
